simulink model "mdltext"  (R2027a)
settings: Solver=VariableStepAuto
model workspace (MAT data in the model file):
  cfg.mode = 'fast'
  cfg.gain = 2
  flag = 1
  gainP = Simulink.Parameter
  gainP.Value = 2.5
  gainP.Complexity = 'real'
  gainP.Dimensions = [1 1]
  gainP.Description = 'gain'
  grid = [1  2  3; 4  5  6]
  inner = -3
  label = 'hello'
  names = {'alpha', 'beta'}
  tau = 0.25
undefined symbols (not defined in the file): Kp
settings Model: DataDictionary=mdltextparams.sldd

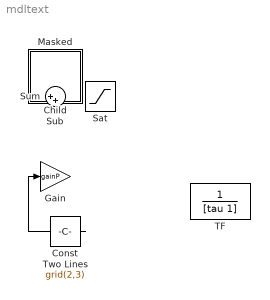
== system mdltext ==
  Child : ModelReference  ZOffset=4  ModelNameDialog=mdltext_child  ModelReferenceVersion=1.1
  Const : Constant  Value=Kp
  Gain : Gain  Gain=gainP
  Masked : Subsystem  ZOffset=3  IfSwitchCaseConditionIndex=0  mask{g=cfg.gain, mode=label}
      mask TypeOptions mode: label | other
  Sat : Saturate  UpperLimit=Inf  LowerLimit=-Inf
  Sub : Subsystem  ZOffset=2  IfSwitchCaseConditionIndex=0
  Sum : Sum  Inputs=|++
  TF : TransferFcn  Denominator=[tau 1]
  Two Lines : Constant  ZOffset=1  Value=grid(2,3)
  wires:
  Const/1 -> Gain/1

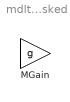
== system mdltext/Masked ==
  MGain : Gain  Gain=g

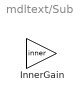
== system mdltext/Sub ==
  InnerGain : Gain  Gain=inner
